simulink model "cable_driven_parallel_robot2022"  (R2022b)
settings: Solver=ode3  StartTime=0.0  StopTime=100  FixedStep=0.01  RelTol=1e-3
values from neighbouring files (symbols this model uses):
  cable_length = 1.2    [Model_Info.m]
  g = 9.81    [Model_Info.m]
  MP_H = 2    [Model_Info.m]
  MP_init_X = 0    [Model_Info.m]
  MP_init_Y = 0    [Model_Info.m]
  MP_init_Z = cable_length + (MP_H/2)    (= 2.2)    [Model_Info.m]
  MP_Ix = (MP_m/12)*(MP_W^2+MP_H^2)    (= 6.66666666667e-05)    [Model_Info.m]
  MP_Iy = (MP_m/12)*(MP_L^2+MP_H^2)    (= 6.66666666667e-05)    [Model_Info.m]
  MP_Iz = (MP_m/12)*(MP_L^2+MP_W^2)    (= 6.66666666667e-05)    [Model_Info.m]
  MP_L = 2    [Model_Info.m]
  MP_m = 0.0001    [Model_Info.m]
  MP_W = 2    [Model_Info.m]
  MR_init_X_L1 = -(MP_L/2)    (= -1)    [Model_Info.m]
  MR_init_X_L2 = (MP_L/2)    (= 1)    [Model_Info.m]
  MR_init_X_L3 = (MP_L/2)    (= 1)    [Model_Info.m]
  MR_init_X_L4 = -(MP_L/2)    (= -1)    [Model_Info.m]
  MR_init_Y_L1 = -(MP_W/2)    (= -1)    [Model_Info.m]
  MR_init_Y_L2 = -(MP_W/2)    (= -1)    [Model_Info.m]
  MR_init_Y_L3 = (MP_W/2)    (= 1)    [Model_Info.m]
  MR_init_Y_L4 = (MP_W/2)    (= 1)    [Model_Info.m]
  MR_init_Yaw_L1 = pi    (= 3.14159265359)    [Model_Info.m]
  MR_init_Yaw_L2 = 0    [Model_Info.m]
  MR_init_Yaw_L3 = 0    [Model_Info.m]
  MR_init_Yaw_L4 = pi    (= 3.14159265359)    [Model_Info.m]
  MR_Jr = (MR_m/12)*(MR_L^2+MR_W^2)    (= 0.333333333333)    [Model_Info.m]
  MR_m = 0.5    [Model_Info.m]
  MR_r = 2    [Model_Info.m]
  MR_WT = 2    [Model_Info.m]
  QR_Ax = 0.25*0    (= 0)    [Model_Info.m]
  QR_Ay = 0.25*0    (= 0)    [Model_Info.m]
  QR_Az = 0.25*0    (= 0)    [Model_Info.m]
  QR_b = 1.14*1e-7    (= 1.14e-07)    [Model_Info.m]
  QR_Ixx = 4.856*1e-3    (= 0.004856)    [Model_Info.m]
  QR_Iyy = 4.856*1e-3    (= 0.004856)    [Model_Info.m]
  QR_Izz = 8.801*1e-3    (= 0.008801)    [Model_Info.m]
  QR_K = 2.980*1e-6    (= 2.98e-06)    [Model_Info.m]
  QR_l = 0.225    [Model_Info.m]
  QR_m = 0.468    [Model_Info.m]
  QR_x0_U1 = -(MP_L/2)    (= -1)    [Model_Info.m]
  QR_x0_U2 = (MP_L/2)    (= 1)    [Model_Info.m]
  QR_x0_U3 = (MP_L/2)    (= 1)    [Model_Info.m]
  QR_x0_U4 = -(MP_L/2)    (= -1)    [Model_Info.m]
  QR_y0_U1 = -(MP_W/2)    (= -1)    [Model_Info.m]
  QR_y0_U2 = -(MP_W/2)    (= -1)    [Model_Info.m]
  QR_y0_U3 = (MP_W/2)    (= 1)    [Model_Info.m]
  QR_y0_U4 = (MP_W/2)    (= 1)    [Model_Info.m]
  QR_z0_U1 = 2*cable_length+(MP_H)    (= 4.4)    [Model_Info.m]
  QR_z0_U2 = 2*cable_length+(MP_H)    (= 4.4)    [Model_Info.m]
  QR_z0_U3 = 2*cable_length+(MP_H)    (= 4.4)    [Model_Info.m]
  QR_z0_U4 = 2*cable_length+(MP_H)    (= 4.4)    [Model_Info.m]
(part 12 of 12)

== matlab function cable_driven_parallel_robot2022/Target Wrench-Jacobian matrix/QuadRotor U4/Force Generator/QuadCopter Model ==
  data: vx input; x_ddot output size=1; vy input; vz input; phidot input; thetadot input; psidot input; y_ddot output size=1; z_ddot output size=1; phi input; theta input; psi input; constants input
function [x_ddot,y_ddot,z_ddot] = fcn(vx,vy,vz,phidot,thetadot,psidot, phi,theta,psi,constants)
m = constants(1);
g = constants(2);
Ixx = constants(3);
Iyy = constants(4);
Izz = constants(5);
l = constants(6);
K = constants(7);
b = constants(8);
Ax = constants(9);
Ay = constants(10);
Az = constants(11);
omega1 = constants(12);
omega2 = constants(13);
omega3 = constants(14);
omega4 = constants(15);
Tx = constants(16);
Ty = constants(17);
Tz = constants(18);
% x_ddot = (K*omega1^2*sin(phi)*sin(psi) - Ax*vx + K*omega2^2*sin(phi)*sin(psi) + K*omega3^2*sin(phi)*sin(psi) + K*omega4^2*sin(phi)*sin(psi) + K*omega1^2*cos(phi)*cos(psi)*sin(theta) + K*omega2^2*cos(phi)*cos(psi)*sin(theta) + K*omega3^2*cos(phi)*cos(psi)*sin(theta) + K*omega4^2*cos(phi)*cos(psi)*sin(theta))/m;
% y_ddot = -(Ay*vy + K*omega1^2*cos(psi)*sin(phi) + K*omega2^2*cos(psi)*sin(phi) + K*omega3^2*cos(psi)*sin(phi) + K*omega4^2*cos(psi)*sin(phi) - K*omega1^2*cos(phi)*sin(psi)*sin(theta) - K*omega2^2*cos(phi)*sin(psi)*sin(theta) - K*omega3^2*cos(phi)*sin(psi)*sin(theta) - K*omega4^2*cos(phi)*sin(psi)*sin(theta))/m;
% z_ddot = (K*cos(phi)*cos(theta)*omega1^2 + K*cos(phi)*cos(theta)*omega2^2 + K*cos(phi)*cos(theta)*omega3^2 + K*cos(phi)*cos(theta)*omega4^2 - Az*vz - g*m)/m;
% phi_ddot = (2*Ixx*Iyy*b*omega1^2*sin(theta) - 2*Ixx*Iyy*b*omega2^2*sin(theta) + 2*Ixx*Iyy*b*omega3^2*sin(theta) - 2*Ixx*Iyy*b*omega4^2*sin(theta) + 2*Iyy^3*psidot^2*cos(phi)*cos(theta)^4*sin(phi)^3 - 2*Iyy^3*psidot^2*cos(phi)*cos(theta)^4*sin(phi)^5 - 2*Iyy^3*psidot*thetadot*cos(theta)^3*sin(phi)^2 + 2*Iyy^3*psidot*thetadot*cos(theta)^3*sin(phi)^4 - 2*Iyy^3*psidot^2*cos(phi)^3*cos(theta)^4*sin(phi)^3 - Iyy^3*thetadot^2*sin(2*phi)*cos(theta)^2*sin(phi)^2 + Iyy^3*thetadot^2*sin(2*phi)*cos(theta)^2*sin(phi)^4 - Ixx*Iyy^2*thetadot^2*sin(2*phi)*sin(theta)^2 - 2*Iyy^2*K*l*omega2^2*cos(theta)^2*sin(phi)^2 + 2*Iyy^2*K*l*omega2^2*cos(theta)^2*sin(phi)^4 + 2*Iyy^2*K*l*omega4^2*cos(theta)^2*sin(phi)^2 - 2*Iyy^2*K*l*omega4^2*cos(theta)^2*sin(phi)^4 + 2*Ixx*Iyy^2*thetadot^2*cos(phi)*sin(phi)*sin(theta)^2 - 2*Ixx*Iyy*b*omega1^2*sin(phi)^2*sin(theta) + 2*Ixx*Iyy*b*omega2^2*sin(phi)^2*sin(theta) - 2*Ixx*Iyy*b*omega3^2*sin(phi)^2*sin(theta) + 2*Ixx*Iyy*b*omega4^2*sin(phi)^2*sin(theta) + 2*Ixx*Izz*b*omega1^2*sin(phi)^2*sin(theta) - 2*Ixx*Izz*b*omega2^2*sin(phi)^2*sin(theta) + 2*Ixx*Izz*b*omega3^2*sin(phi)^2*sin(theta) - 2*Ixx*Izz*b*omega4^2*sin(phi)^2*sin(theta) - 2*Ixx*Iyy^2*psidot*thetadot*cos(theta)*sin(theta)^2 + 2*Ixx^2*Iyy*psidot*thetadot*cos(theta)*sin(theta)^2 + 2*Ixx*Iyy^2*psidot*thetadot*sin(2*theta)*sin(theta) - 2*Ixx^2*Iyy*psidot*thetadot*sin(2*theta)*sin(theta) - 2*Iyy*Izz^2*psidot^2*cos(phi)^3*cos(theta)^4*sin(phi) - 2*Iyy^2*Izz*psidot^2*cos(phi)*cos(theta)^4*sin(phi)^3 + 2*Iyy^2*Izz*psidot^2*cos(phi)^3*cos(theta)^4*sin(phi) - 2*Iyy*Izz^2*psidot^2*cos(phi)*cos(theta)^4*sin(phi)^5 + 4*Iyy^2*Izz*psidot^2*cos(phi)*cos(theta)^4*sin(phi)^5 - 2*Ixx*Iyy^2*thetadot^2*cos(phi)*sin(phi)^3*sin(theta)^2 - 2*Ixx*Izz^2*thetadot^2*cos(phi)*sin(phi)^3*sin(theta)^2 + Ixx*Iyy*Izz*thetadot^2*sin(2*phi)*sin(theta)^2 + 6*Iyy^3*psidot*thetadot*cos(phi)^2*cos(theta)^3*sin(phi)^2 - 4*Iyy^3*psidot*thetadot*cos(phi)^2*cos(theta)^3*sin(phi)^4 - 4*Iyy^3*psidot*thetadot*cos(phi)^4*cos(theta)^3*sin(phi)^2 + 2*Iyy*Izz^2*psidot*thetadot*cos(phi)^2*cos(theta)^3 - 2*Iyy^2*Izz*psidot*thetadot*cos(phi)^2*cos(theta)^3 - 4*Iyy*Izz^2*psidot*thetadot*cos(phi)^4*cos(theta)^3 + 4*Iyy^2*Izz*psidot*thetadot*cos(phi)^4*cos(theta)^3 + 2*Ixx*Iyy^2*psidot*thetadot*cos(theta)^3*sin(phi)^2 - 2*Ixx*Iyy^2*psidot*thetadot*cos(theta)^3*sin(phi)^4 + 2*Iyy^2*Izz*psidot*thetadot*cos(theta)^3*sin(phi)^2 + 2*Iyy*Izz^2*psidot*thetadot*cos(theta)^3*sin(phi)^4 - 4*Iyy^2*Izz*psidot*thetadot*cos(theta)^3*sin(phi)^4 - 2*Ixx*Iyy*K*l*omega2^2*sin(theta)^2 + 2*Ixx*Iyy*K*l*omega4^2*sin(theta)^2 + Iyy^3*thetadot^2*sin(2*phi)*cos(phi)^2*cos(theta)^2*sin(phi)^2 - 2*Iyy*Izz^2*psidot^2*cos(phi)^3*cos(theta)^4*sin(phi)^3 + 4*Iyy^2*Izz*psidot^2*cos(phi)^3*cos(theta)^4*sin(phi)^3 + Iyy*Izz^2*thetadot^2*sin(2*phi)*cos(phi)^2*cos(theta)^2 - Iyy^2*Izz*thetadot^2*sin(2*phi)*cos(phi)^2*cos(theta)^2 + Iyy^2*Izz*thetadot^2*sin(2*phi)*cos(theta)^2*sin(phi)^2 + Iyy*Izz^2*thetadot^2*sin(2*phi)*cos(theta)^2*sin(phi)^4 - 2*Iyy^2*Izz*thetadot^2*sin(2*phi)*cos(theta)^2*sin(phi)^4 + Ixx*Iyy^2*thetadot^2*sin(2*phi)*sin(phi)^2*sin(theta)^2 + Ixx*Izz^2*thetadot^2*sin(2*phi)*sin(phi)^2*sin(theta)^2 + 2*Ixx*Iyy^2*phidot*thetadot*cos(theta)*sin(theta) + 2*Ixx^2*Iyy*phidot*thetadot*cos(theta)*sin(theta) + 2*Ixx*Iyy*K*l*omega2^2*sin(phi)^2*sin(theta)^2 - 2*Ixx*Iyy*K*l*omega4^2*sin(phi)^2*sin(theta)^2 - 2*Ixx*Izz*K*l*omega2^2*sin(phi)^2*sin(theta)^2 + 2*Ixx*Izz*K*l*omega4^2*sin(phi)^2*sin(theta)^2 - 2*Ixx*Iyy*Izz*thetadot^2*cos(phi)*sin(phi)*sin(theta)^2 + Iyy*Izz^2*thetadot^2*sin(2*phi)*cos(phi)^2*cos(theta)^2*sin(phi)^2 - 2*Iyy^2*Izz*thetadot^2*sin(2*phi)*cos(phi)^2*cos(theta)^2*sin(phi)^2 - 4*Ixx*Iyy^2*phidot*thetadot*cos(phi)^2*cos(theta)*sin(theta) - 2*Ixx*Iyy^2*phidot*thetadot*cos(theta)*sin(phi)^2*sin(theta) - 2*Ixx^2*Iyy*phidot*thetadot*cos(theta)*sin(phi)^2*sin(theta) - 2*Ixx*Izz^2*phidot*thetadot*cos(theta)*sin(phi)^2*sin(theta) + 2*Ixx^2*Izz*phidot*thetadot*cos(theta)*sin(phi)^2*sin(theta) + 2*Iyy^2*K*l*omega2^2*cos(phi)^2*cos(theta)^2*sin(phi)^2 - 2*Iyy^2*K*l*omega4^2*cos(phi)^2*cos(theta)^2*sin(phi)^2 + 2*Ixx*Iyy*Izz*psidot*thetadot*cos(theta)*sin(theta)^2 + 2*Ixx*Iyy^2*psidot^2*cos(phi)*cos(theta)^2*sin(phi)*sin(theta)^2 + 4*Ixx*Iyy*Izz*thetadot^2*cos(phi)*sin(phi)^3*sin(theta)^2 + 2*Ixx*Iyy*Izz*psidot*thetadot*cos(phi)^2*cos(theta)^3 + 2*Ixx*Iyy^2*psidot*thetadot*cos(theta)*sin(phi)^2*sin(theta)^2 - 2*Ixx^2*Iyy*psidot*thetadot*cos(theta)*sin(phi)^2*sin(theta)^2 + 2*Ixx*Izz^2*psidot*thetadot*cos(theta)*sin(phi)^2*sin(theta)^2 + 2*Ixx^2*Izz*psidot*thetadot*cos(theta)*sin(phi)^2*sin(theta)^2 + 2*Ixx*Iyy*Izz*psidot*thetadot*cos(theta)^3*sin(phi)^4 - 2*Ixx*Iyy^2*psidot*thetadot*sin(2*theta)*sin(phi)^2*sin(theta) + 2*Ixx^2*Iyy*psidot*thetadot*sin(2*theta)*sin(phi)^2*sin(theta) - 2*Ixx^2*Izz*psidot*thetadot*sin(2*theta)*sin(phi)^2*sin(theta) - 2*Ixx*Izz^2*psidot^2*cos(phi)*cos(theta)^2*sin(phi)^3*sin(theta)^2 - 2*Ixx*Izz^2*psidot^2*cos(phi)^3*cos(theta)^2*sin(phi)*sin(theta)^2 - 2*Ixx*Iyy*Izz*thetadot^2*sin(2*phi)*sin(phi)^2*sin(theta)^2 - 2*Ixx*Iyy*Izz*phidot*thetadot*cos(theta)*sin(theta) - 2*Iyy*Izz*K*l*omega2^2*cos(phi)^2*cos(theta)^2 + 2*Iyy*Izz*K*l*omega4^2*cos(phi)^2*cos(theta)^2 - 2*Ixx*Iyy^2*psidot*thetadot*cos(phi)^2*cos(theta)^3*sin(phi)^2 + 2*Iyy*Izz^2*psidot*thetadot*cos(phi)^2*cos(theta)^3*sin(phi)^2 - 8*Iyy^2*Izz*psidot*thetadot*cos(phi)^2*cos(theta)^3*sin(phi)^2 - 4*Iyy*Izz^2*psidot*thetadot*cos(phi)^2*cos(theta)^3*sin(phi)^4 - 4*Iyy*Izz^2*psidot*thetadot*cos(phi)^4*cos(theta)^3*sin(phi)^2 + 8*Iyy^2*Izz*psidot*thetadot*cos(phi)^2*cos(theta)^3*sin(phi)^4 + 8*Iyy^2*Izz*psidot*thetadot*cos(phi)^4*cos(theta)^3*sin(phi)^2 - 2*Iyy*Izz*K*l*omega2^2*cos(theta)^2*sin(phi)^4 + 2*Iyy*Izz*K*l*omega4^2*cos(theta)^2*sin(phi)^4 - 4*Ixx*Iyy^2*phidot*psidot*cos(phi)*cos(theta)^2*sin(phi)*sin(theta) + 2*Ixx^2*Iyy*phidot*psidot*cos(phi)*cos(theta)^2*sin(phi)*sin(theta) - 2*Ixx^2*Izz*phidot*psidot*cos(phi)*cos(theta)^2*sin(phi)*sin(theta) + 4*Ixx*Iyy*Izz*phidot*thetadot*cos(phi)^2*cos(theta)*sin(theta) + 4*Ixx*Iyy*Izz*phidot*thetadot*cos(theta)*sin(phi)^2*sin(theta) - 2*Iyy*Izz*K*l*omega2^2*cos(phi)^2*cos(theta)^2*sin(phi)^2 + 2*Iyy*Izz*K*l*omega4^2*cos(phi)^2*cos(theta)^2*sin(phi)^2 - 2*Ixx*Iyy*Izz*psidot^2*cos(phi)*cos(theta)^2*sin(phi)*sin(theta)^2 + 2*Ixx*Iyy^2*phidot*psidot*cos(phi)*cos(theta)^2*sin(phi)^3*sin(theta) + 2*Ixx*Iyy^2*phidot*psidot*cos(phi)^3*cos(theta)^2*sin(phi)*sin(theta) + 2*Ixx*Izz^2*phidot*psidot*cos(phi)*cos(theta)^2*sin(phi)^3*sin(theta) + 2*Ixx*Izz^2*phidot*psidot*cos(phi)^3*cos(theta)^2*sin(phi)*sin(theta) + 4*Ixx*Iyy^2*phidot*thetadot*cos(phi)^2*cos(theta)*sin(phi)^2*sin(theta) + 4*Ixx*Izz^2*phidot*thetadot*cos(phi)^2*cos(theta)*sin(phi)^2*sin(theta) - 4*Ixx*Iyy*Izz*psidot*thetadot*cos(theta)*sin(phi)^2*sin(theta)^2 + 2*Ixx*Iyy*Izz*psidot*thetadot*sin(2*theta)*sin(phi)^2*sin(theta) + 2*Ixx*Iyy*Izz*psidot^2*cos(phi)*cos(theta)^2*sin(phi)^3*sin(theta)^2 + 2*Ixx*Iyy*Izz*psidot^2*cos(phi)^3*cos(theta)^2*sin(phi)*sin(theta)^2 + 2*Ixx*Iyy*Izz*psidot*thetadot*cos(phi)^2*cos(theta)^3*sin(phi)^2 - Ixx^2*Iyy*psidot^2*sin(2*theta)*cos(phi)*cos(theta)*sin(phi)*sin(theta) + Ixx^2*Izz*psidot^2*sin(2*theta)*cos(phi)*cos(theta)*sin(phi)*sin(theta) - 4*Ixx*Iyy*Izz*phidot*psidot*cos(phi)*cos(theta)^2*sin(phi)^3*sin(theta) - 4*Ixx*Iyy*Izz*phidot*psidot*cos(phi)^3*cos(theta)^2*sin(phi)*sin(theta) - 8*Ixx*Iyy*Izz*phidot*thetadot*cos(phi)^2*cos(theta)*sin(phi)^2*sin(theta) + 2*Ixx*Iyy*K*l*omega1^2*cos(phi)*cos(theta)*sin(phi)*sin(theta) - 2*Ixx*Iyy*K*l*omega3^2*cos(phi)*cos(theta)*sin(phi)*sin(theta) - 2*Ixx*Izz*K*l*omega1^2*cos(phi)*cos(theta)*sin(phi)*sin(theta) + 2*Ixx*Izz*K*l*omega3^2*cos(phi)*cos(theta)*sin(phi)*sin(theta) - 2*Ixx*Iyy^2*phidot*thetadot*sin(2*phi)*cos(phi)*cos(theta)*sin(phi)*sin(theta) - 2*Ixx*Izz^2*phidot*thetadot*sin(2*phi)*cos(phi)*cos(theta)*sin(phi)*sin(theta) + 4*Ixx*Iyy*Izz*phidot*psidot*cos(phi)*cos(theta)^2*sin(phi)*sin(theta) + 4*Ixx*Iyy*Izz*phidot*thetadot*sin(2*phi)*cos(phi)*cos(theta)*sin(phi)*sin(theta))/(2*Ixx*cos(theta)^2*(- Iyy^2*cos(phi)^2*sin(phi)^2 - Iyy^2*sin(phi)^4 + Iyy^2*sin(phi)^2 + Izz*Iyy*cos(phi)^2*sin(phi)^2 + Izz*Iyy*cos(phi)^2 + Izz*Iyy*sin(phi)^4));
% theta_ddot = -(2*Izz^2*psidot^2*cos(phi)^4*cos(theta)^2*sin(theta) + 2*Iyy^2*thetadot^2*cos(phi)^2*sin(phi)^2*sin(theta) + 2*Izz^2*thetadot^2*cos(phi)^2*sin(phi)^2*sin(theta) + 2*Iyy^2*psidot^2*cos(theta)^2*sin(phi)^4*sin(theta) - 2*Izz^2*phidot*psidot*cos(phi)^4*cos(theta)^2 - 2*Iyy^2*phidot*psidot*cos(theta)^2*sin(phi)^4 + 2*Iyy*b*omega1^2*cos(phi)*sin(phi) - 2*Iyy*b*omega2^2*cos(phi)*sin(phi) + 2*Iyy*b*omega3^2*cos(phi)*sin(phi) - 2*Iyy*b*omega4^2*cos(phi)*sin(phi) - 2*Izz*b*omega1^2*cos(phi)*sin(phi) + 2*Izz*b*omega2^2*cos(phi)*sin(phi) - 2*Izz*b*omega3^2*cos(phi)*sin(phi) + 2*Izz*b*omega4^2*cos(phi)*sin(phi) - Ixx*Izz*psidot^2*sin(2*theta)*cos(phi)^2*cos(theta) - 4*Iyy*Izz*thetadot^2*cos(phi)^2*sin(phi)^2*sin(theta) - Ixx*Iyy*psidot^2*sin(2*theta)*cos(theta)*sin(phi)^2 + 2*Izz*K*l*omega1^2*cos(phi)^2*cos(theta) - 2*Izz*K*l*omega3^2*cos(phi)^2*cos(theta) + 2*Izz^2*phidot*thetadot*sin(2*phi)*cos(phi)^2*cos(theta) + 2*Ixx*Izz*phidot*psidot*cos(phi)^2*cos(theta)^2 + 2*Iyy*Izz*phidot*psidot*cos(phi)^4*cos(theta)^2 + 2*Iyy*K*l*omega1^2*cos(theta)*sin(phi)^2 - 2*Iyy*K*l*omega3^2*cos(theta)*sin(phi)^2 - 2*Iyy^2*phidot*thetadot*sin(2*phi)*cos(theta)*sin(phi)^2 + 2*Ixx*Iyy*phidot*psidot*cos(theta)^2*sin(phi)^2 + 2*Iyy*Izz*phidot*psidot*cos(theta)^2*sin(phi)^4 + 2*Iyy^2*psidot^2*cos(phi)^2*cos(theta)^2*sin(phi)^2*sin(theta) + 2*Izz^2*psidot^2*cos(phi)^2*cos(theta)^2*sin(phi)^2*sin(theta) + 2*Iyy^2*phidot*thetadot*cos(phi)*cos(theta)*sin(phi) + 2*Izz^2*phidot*thetadot*cos(phi)*cos(theta)*sin(phi) - 2*Iyy^2*phidot*psidot*cos(phi)^2*cos(theta)^2*sin(phi)^2 - 2*Izz^2*phidot*psidot*cos(phi)^2*cos(theta)^2*sin(phi)^2 - Iyy^2*thetadot^2*sin(2*phi)*cos(phi)*sin(phi)*sin(theta) - Izz^2*thetadot^2*sin(2*phi)*cos(phi)*sin(phi)*sin(theta) - 4*Iyy^2*phidot*thetadot*cos(phi)^3*cos(theta)*sin(phi) - 4*Izz^2*phidot*thetadot*cos(phi)^3*cos(theta)*sin(phi) + 2*Iyy^2*psidot*thetadot*sin(2*theta)*cos(phi)*sin(phi) - 2*Iyy*Izz*phidot*thetadot*sin(2*phi)*cos(phi)^2*cos(theta) + 2*Iyy*Izz*phidot*thetadot*sin(2*phi)*cos(theta)*sin(phi)^2 - 2*Iyy^2*psidot*thetadot*cos(phi)*cos(theta)*sin(phi)*sin(theta) - 2*Izz^2*psidot*thetadot*cos(phi)*cos(theta)*sin(phi)*sin(theta) + 2*Ixx*Iyy*phidot*thetadot*cos(phi)*cos(theta)*sin(phi) - 2*Ixx*Izz*phidot*thetadot*cos(phi)*cos(theta)*sin(phi) - 4*Iyy*Izz*phidot*thetadot*cos(phi)*cos(theta)*sin(phi) + 4*Iyy*Izz*phidot*psidot*cos(phi)^2*cos(theta)^2*sin(phi)^2 + 2*Iyy*Izz*thetadot^2*sin(2*phi)*cos(phi)*sin(phi)*sin(theta) + 8*Iyy*Izz*phidot*thetadot*cos(phi)^3*cos(theta)*sin(phi) - 2*Iyy*K*l*omega2^2*cos(phi)*sin(phi)*sin(theta) + 2*Iyy*K*l*omega4^2*cos(phi)*sin(phi)*sin(theta) + 2*Izz*K*l*omega2^2*cos(phi)*sin(phi)*sin(theta) - 2*Izz*K*l*omega4^2*cos(phi)*sin(phi)*sin(theta) - 2*Ixx*Iyy*psidot*thetadot*sin(2*theta)*cos(phi)*sin(phi) + 2*Ixx*Izz*psidot*thetadot*sin(2*theta)*cos(phi)*sin(phi) - 2*Iyy*Izz*psidot*thetadot*sin(2*theta)*cos(phi)*sin(phi) + 2*Ixx*Iyy*psidot*thetadot*cos(phi)*cos(theta)*sin(phi)*sin(theta) - 2*Ixx*Izz*psidot*thetadot*cos(phi)*cos(theta)*sin(phi)*sin(theta) + 4*Iyy*Izz*psidot*thetadot*cos(phi)*cos(theta)*sin(phi)*sin(theta))/(2*cos(theta)*(- Iyy^2*cos(phi)^2*sin(phi)^2 - Iyy^2*sin(phi)^4 + Iyy^2*sin(phi)^2 + Izz*Iyy*cos(phi)^2*sin(phi)^2 + Izz*Iyy*cos(phi)^2 + Izz*Iyy*sin(phi)^4));
% psi_ddot = (2*Iyy*b*omega1^2 - 2*Iyy*b*omega2^2 + 2*Iyy*b*omega3^2 - 2*Iyy*b*omega4^2 - Iyy^2*thetadot^2*sin(2*phi)*sin(theta) - 2*Iyy*b*omega1^2*sin(phi)^2 + 2*Iyy*b*omega2^2*sin(phi)^2 - 2*Iyy*b*omega3^2*sin(phi)^2 + 2*Iyy*b*omega4^2*sin(phi)^2 + 2*Izz*b*omega1^2*sin(phi)^2 - 2*Izz*b*omega2^2*sin(phi)^2 + 2*Izz*b*omega3^2*sin(phi)^2 - 2*Izz*b*omega4^2*sin(phi)^2 + 2*Iyy^2*psidot*thetadot*sin(2*theta) + 2*Iyy^2*phidot*thetadot*cos(theta) - 2*Iyy^2*phidot*thetadot*cos(theta)*sin(phi)^2 - 2*Izz^2*phidot*thetadot*cos(theta)*sin(phi)^2 - 2*Iyy*K*l*omega2^2*sin(theta) + 2*Iyy*K*l*omega4^2*sin(theta) - 2*Ixx*Iyy*psidot*thetadot*sin(2*theta) + Iyy^2*thetadot^2*sin(2*phi)*sin(phi)^2*sin(theta) + Izz^2*thetadot^2*sin(2*phi)*sin(phi)^2*sin(theta) - 2*Iyy^2*psidot*thetadot*sin(2*theta)*sin(phi)^2 + 2*Iyy^2*thetadot^2*cos(phi)*sin(phi)*sin(theta) - 2*Iyy^2*psidot*thetadot*cos(theta)*sin(theta) + 2*Ixx*Iyy*phidot*thetadot*cos(theta) - 2*Iyy*Izz*phidot*thetadot*cos(theta) - 2*Iyy^2*thetadot^2*cos(phi)*sin(phi)^3*sin(theta) - 2*Izz^2*thetadot^2*cos(phi)*sin(phi)^3*sin(theta) + Iyy*Izz*thetadot^2*sin(2*phi)*sin(theta) - 4*Iyy^2*phidot*thetadot*cos(phi)^2*cos(theta) - 2*Izz^2*psidot^2*cos(phi)*cos(theta)^2*sin(phi)^3*sin(theta) - 2*Izz^2*psidot^2*cos(phi)^3*cos(theta)^2*sin(phi)*sin(theta) - 2*Iyy*Izz*thetadot^2*sin(2*phi)*sin(phi)^2*sin(theta) + 2*Iyy^2*phidot*psidot*cos(phi)*cos(theta)^2*sin(phi)^3 + 2*Iyy^2*phidot*psidot*cos(phi)^3*cos(theta)^2*sin(phi) + 2*Izz^2*phidot*psidot*cos(phi)*cos(theta)^2*sin(phi)^3 + 2*Izz^2*phidot*psidot*cos(phi)^3*cos(theta)^2*sin(phi) + 4*Iyy^2*phidot*thetadot*cos(phi)^2*cos(theta)*sin(phi)^2 + 4*Izz^2*phidot*thetadot*cos(phi)^2*cos(theta)*sin(phi)^2 + 2*Iyy*K*l*omega2^2*sin(phi)^2*sin(theta) - 2*Iyy*K*l*omega4^2*sin(phi)^2*sin(theta) - 2*Izz*K*l*omega2^2*sin(phi)^2*sin(theta) + 2*Izz*K*l*omega4^2*sin(phi)^2*sin(theta) + 2*Ixx*Iyy*psidot*thetadot*sin(2*theta)*sin(phi)^2 - 2*Ixx*Izz*psidot*thetadot*sin(2*theta)*sin(phi)^2 + 2*Iyy*Izz*psidot*thetadot*sin(2*theta)*sin(phi)^2 - 2*Iyy*Izz*thetadot^2*cos(phi)*sin(phi)*sin(theta) + 2*Ixx*Iyy*psidot*thetadot*cos(theta)*sin(theta) + 2*Iyy*Izz*psidot*thetadot*cos(theta)*sin(theta) + 2*Iyy^2*psidot^2*cos(phi)*cos(theta)^2*sin(phi)*sin(theta) + 4*Iyy*Izz*thetadot^2*cos(phi)*sin(phi)^3*sin(theta) - 4*Iyy^2*phidot*psidot*cos(phi)*cos(theta)^2*sin(phi) + 4*Iyy*Izz*phidot*thetadot*cos(phi)^2*cos(theta) + 2*Iyy^2*psidot*thetadot*cos(theta)*sin(phi)^2*sin(theta) + 2*Izz^2*psidot*thetadot*cos(theta)*sin(phi)^2*sin(theta) - 2*Ixx*Iyy*phidot*thetadot*cos(theta)*sin(phi)^2 + 2*Ixx*Izz*phidot*thetadot*cos(theta)*sin(phi)^2 + 4*Iyy*Izz*phidot*thetadot*cos(theta)*sin(phi)^2 - 4*Iyy*Izz*phidot*psidot*cos(phi)*cos(theta)^2*sin(phi)^3 - 4*Iyy*Izz*phidot*psidot*cos(phi)^3*cos(theta)^2*sin(phi) - 8*Iyy*Izz*phidot*thetadot*cos(phi)^2*cos(theta)*sin(phi)^2 - Ixx*Iyy*psidot^2*sin(2*theta)*cos(phi)*cos(theta)*sin(phi) + Ixx*Izz*psidot^2*sin(2*theta)*cos(phi)*cos(theta)*sin(phi) - 2*Iyy*Izz*psidot^2*cos(phi)*cos(theta)^2*sin(phi)*sin(theta) + 2*Iyy*K*l*omega1^2*cos(phi)*cos(theta)*sin(phi) - 2*Iyy*K*l*omega3^2*cos(phi)*cos(theta)*sin(phi) - 2*Izz*K*l*omega1^2*cos(phi)*cos(theta)*sin(phi) + 2*Izz*K*l*omega3^2*cos(phi)*cos(theta)*sin(phi) - 2*Iyy^2*phidot*thetadot*sin(2*phi)*cos(phi)*cos(theta)*sin(phi) - 2*Izz^2*phidot*thetadot*sin(2*phi)*cos(phi)*cos(theta)*sin(phi) + 2*Ixx*Iyy*phidot*psidot*cos(phi)*cos(theta)^2*sin(phi) - 2*Ixx*Izz*phidot*psidot*cos(phi)*cos(theta)^2*sin(phi) + 4*Iyy*Izz*phidot*psidot*cos(phi)*cos(theta)^2*sin(phi) - 2*Ixx*Iyy*psidot*thetadot*cos(theta)*sin(phi)^2*sin(theta) + 2*Ixx*Izz*psidot*thetadot*cos(theta)*sin(phi)^2*sin(theta) - 4*Iyy*Izz*psidot*thetadot*cos(theta)*sin(phi)^2*sin(theta) + 2*Iyy*Izz*psidot^2*cos(phi)*cos(theta)^2*sin(phi)^3*sin(theta) + 2*Iyy*Izz*psidot^2*cos(phi)^3*cos(theta)^2*sin(phi)*sin(theta) + 4*Iyy*Izz*phidot*thetadot*sin(2*phi)*cos(phi)*cos(theta)*sin(phi))/(2*cos(theta)^2*(- Iyy^2*cos(phi)^2*sin(phi)^2 - Iyy^2*sin(phi)^4 + Iyy^2*sin(phi)^2 + Izz*Iyy*cos(phi)^2*sin(phi)^2 + Izz*Iyy*cos(phi)^2 + Izz*Iyy*sin(phi)^4));
x_ddot =  (K*omega1^2*sin(phi)*sin(psi) - Ax*vx - Tx + K*omega2^2*sin(phi)*sin(psi) + K*omega3^2*sin(phi)*sin(psi) + K*omega4^2*sin(phi)*sin(psi) + K*omega1^2*cos(phi)*cos(psi)*sin(theta) + K*omega2^2*cos(phi)*cos(psi)*sin(theta) + K*omega3^2*cos(phi)*cos(psi)*sin(theta) + K*omega4^2*cos(phi)*cos(psi)*sin(theta))/m;
y_ddot = -(Ty + Ay*vy + K*omega1^2*cos(psi)*sin(phi) + K*omega2^2*cos(psi)*sin(phi) + K*omega3^2*cos(psi)*sin(phi) + K*omega4^2*cos(psi)*sin(phi) - K*omega1^2*cos(phi)*sin(psi)*sin(theta) - K*omega2^2*cos(phi)*sin(psi)*sin(theta) - K*omega3^2*cos(phi)*sin(psi)*sin(theta) - K*omega4^2*cos(phi)*sin(psi)*sin(theta))/m;
z_ddot = (K*cos(phi)*cos(theta)*omega1^2 + K*cos(phi)*cos(theta)*omega2^2 + K*cos(phi)*cos(theta)*omega3^2 + K*cos(phi)*cos(theta)*omega4^2 - Tz - Az*vz - g*m)/m;

end

== matlab function cable_driven_parallel_robot2022/Target Wrench-Jacobian matrix/Moving Platform/Moving Platform/QR Force Generator ==
  data: mass input; Fx output; Fy output; Fz output
function [Fx,Fy,Fz] = fcn(mass)
g = 9.81;

Fx = 0;
Fy = 0;
Fz = -mass*g; 
    
end

== matlab function cable_driven_parallel_robot2022/Target Wrench-Jacobian matrix/2 Wheels Diffrential Mobile Robot L1/Transform ==
  data: roll input; pitch input; yaw input; MP_X input; MP_Y input; MP_Z input; MP_L1_X output; MP_L1_Y output; MP_L1_Z output; L input; W input; H input
function [MP_L1_X,MP_L1_Y,MP_L1_Z] = fcn(roll,pitch,yaw,MP_X,MP_Y,MP_Z,L,W,H)

MP_C = [1  0  0  MP_X; ... 
        0  1  0  MP_Y; ...
        0  0  1  MP_Z; ...
        0  0  0   1];

R_x = [1      0          0          0; ...
       0  cos(roll) -sin(roll)      0; ...
       0  sin(roll)  cos(roll)      0; ...
       0      0          0          1];
   
R_y = [cos(pitch)  0   sin(pitch)   0; ...
          0        1       0        0; ...
      -sin(pitch)  0   cos(pitch)   0; ...
          0        0       0        1];
   
R_z = [cos(yaw) -sin(yaw)  0        0; ...
       sin(yaw)  cos(yaw)  0        0; ...
         0           0     1        0; ...
         0           0     0        1];

R = MP_C*R_z*R_y*R_x;

Out = R* ([-(L/2);-(W/2) ;-(H/2);1]);
MP_L1_X = Out(1);
MP_L1_Y = Out(2);
MP_L1_Z = Out(3);

== matlab function cable_driven_parallel_robot2022/Target Wrench-Jacobian matrix/2 Wheels Diffrential Mobile Robot L2/Transform ==
  data: roll input; pitch input; yaw input; MP_X input; MP_Y input; MP_Z input; MP_L2_X output; MP_L2_Y output; MP_L2_Z output; L input; W input; H input
function [MP_L2_X,MP_L2_Y,MP_L2_Z] = fcn(roll,pitch,yaw,MP_X,MP_Y,MP_Z,L,W,H)

MP_C = [1  0  0  MP_X; ... 
        0  1  0  MP_Y; ...
        0  0  1  MP_Z; ...
        0  0  0   1];

R_x = [1      0          0          0; ...
       0  cos(roll) -sin(roll)      0; ...
       0  sin(roll)  cos(roll)      0; ...
       0      0          0          1];
   
R_y = [cos(pitch)  0   sin(pitch)   0; ...
          0        1       0        0; ...
      -sin(pitch)  0   cos(pitch)   0; ...
          0        0       0        1];
   
R_z = [cos(yaw) -sin(yaw)  0        0; ...
       sin(yaw)  cos(yaw)  0        0; ...
         0           0     1        0; ...
         0           0     0        1];

R = MP_C*R_z*R_y*R_x;

Out = R* ([(L/2);-(W/2);-(H/2);1]);
MP_L2_X = Out(1);
MP_L2_Y = Out(2);
MP_L2_Z = Out(3);

== matlab function cable_driven_parallel_robot2022/Target Wrench-Jacobian matrix/2 Wheels Diffrential Mobile Robot L3/Transform ==
  data: roll input; pitch input; yaw input; MP_X input; MP_Y input; MP_Z input; MP_L3_X output; MP_L3_Y output; MP_L3_Z output; L input; W input; H input
function [MP_L3_X,MP_L3_Y,MP_L3_Z] = fcn(roll,pitch,yaw,MP_X,MP_Y,MP_Z,L,W,H)

MP_C = [1  0  0  MP_X; ... 
        0  1  0  MP_Y; ...
        0  0  1  MP_Z; ...
        0  0  0   1];

R_x = [1      0          0          0; ...
       0  cos(roll) -sin(roll)      0; ...
       0  sin(roll)  cos(roll)      0; ...
       0      0          0          1];
   
R_y = [cos(pitch)  0   sin(pitch)   0; ...
          0        1       0        0; ...
      -sin(pitch)  0   cos(pitch)   0; ...
          0        0       0        1];
   
R_z = [cos(yaw) -sin(yaw)  0        0; ...
       sin(yaw)  cos(yaw)  0        0; ...
         0           0     1        0; ...
         0           0     0        1];

R = MP_C*R_z*R_y*R_x;

Out = R* ([(L/2);+(W/2);-(H/2);1]);
MP_L3_X = Out(1);
MP_L3_Y = Out(2);
MP_L3_Z = Out(3);

== matlab function cable_driven_parallel_robot2022/Target Wrench-Jacobian matrix/2 Wheels Diffrential Mobile Robot L4/Transform ==
  data: roll input; pitch input; yaw input; MP_X input; MP_Y input; MP_Z input; MP_L4_X output; MP_L4_Y output; MP_L4_Z output; L input; W input; H input
function [MP_L4_X,MP_L4_Y,MP_L4_Z] = fcn(roll,pitch,yaw,MP_X,MP_Y,MP_Z,L,W,H)

MP_C = [1  0  0  MP_X; ... 
        0  1  0  MP_Y; ...
        0  0  1  MP_Z; ...
        0  0  0   1];

R_x = [1      0          0          0; ...
       0  cos(roll) -sin(roll)      0; ...
       0  sin(roll)  cos(roll)      0; ...
       0      0          0          1];
   
R_y = [cos(pitch)  0   sin(pitch)   0; ...
          0        1       0        0; ...
      -sin(pitch)  0   cos(pitch)   0; ...
          0        0       0        1];
   
R_z = [cos(yaw) -sin(yaw)  0        0; ...
       sin(yaw)  cos(yaw)  0        0; ...
         0           0     1        0; ...
         0           0     0        1];

R = MP_C*R_z*R_y*R_x;

Out = R* ([-(L/2);+(W/2);-(H/2);1]);
MP_L4_X = Out(1);
MP_L4_Y = Out(2);
MP_L4_Z = Out(3);

== matlab function cable_driven_parallel_robot2022/Actuators-CableTension-MovingPlatform/Moving Platform/Moving Platform/Moving Platform ==
  settings: updateMethod=DISCRETE
  data: Tx_U1 input; Ty_U1 input; Tz_U1 input; Tx_U2 input; Ty_U2 input; Tz_U2 input; Tx_U3 input; Ty_U3 input; Tz_U3 input; Tx_U4 input; Ty_U4 input; Tz_U4 input; Tx_L1 input; Ty_L1 input; Tz_L1 input; ax output; Tx_L2 input; Ty_L2 input; Tz_L2 input; ay output; Tx_L3 input; Ty_L3 input; Tz_L3 input; Tx_L4 input; Ty_L4 input; Tz_L4 input; m input; Ix input; Iy input; Iz input; gx input; gy input; gz input; L input; W input; H input; az output; alpha_x output; alpha_y output; alpha_z output
function [ax,ay,az,alpha_x,alpha_y,alpha_z] = fcn(Tx_U1,Ty_U1,Tz_U1,Tx_U2,Ty_U2,Tz_U2,Tx_U3,Ty_U3,Tz_U3,Tx_U4,Ty_U4,Tz_U4,Tx_L1,Ty_L1,Tz_L1,Tx_L2,Ty_L2,Tz_L2,Tx_L3,Ty_L3,Tz_L3,Tx_L4,Ty_L4,Tz_L4,m,Ix,Iy,Iz,gx,gy,gz,L,W,H)



ax=(Tx_U1+Tx_U2+Tx_U3+Tx_U4+Tx_L1+Tx_L2+Tx_L3+Tx_L4-m*gx)/m;

ay=(Ty_U1+Ty_U2+Ty_U3+Ty_U4+Ty_L1+Ty_L2+Ty_L3+Ty_L4-m*gy)/m;

az=(Tz_U1+Tz_U2+Tz_U3+Tz_U4+Tz_L1+Tz_L2+Tz_L3+Tz_L4-m*gz)/m;

 alpha_x =((Ty_L1+Ty_L2+Ty_L3+Ty_L4)* (H/2)...
          -(Ty_U1+Ty_U2+Ty_U3+Ty_U4)* (H/2)...
          +(Tz_U3+Tz_U4+Tz_L3+Tz_L4)* (W/2)...
          -(Tz_U1+Tz_U2+Tz_L1+Tz_L2)* (W/2))/Ix;
      
 alpha_y =((Tx_U1+Tx_U2+Tx_U3+Tx_U4)* (H/2)...
          -(Tx_L1+Tx_L2+Tx_L3+Tx_L4)* (H/2)...
          +(Tz_U1+Tz_U4+Tz_L1+Tz_L4)* (L/2)...
          -(Tz_U2+Tz_U3+Tz_L2+Tz_L3)* (L/2))/Iy;
      
 alpha_z =((Tx_U1+Tx_U2+Tx_L1+Tx_L2)* (W/2)...
          -(Tx_U3+Tx_U4+Tx_L3+Tx_L4)* (W/2)...
          +(Ty_U2+Ty_U3+Ty_L2+Ty_L3)* (L/2)...
          -(Ty_U1+Ty_U4+Ty_L1+Ty_L4)* (L/2))/Iz;

== matlab function cable_driven_parallel_robot2022/Target Wrench-Jacobian matrix/QuadRotor U1/Transform ==
  data: roll input; pitch input; yaw input; MP_X input; MP_Y input; MP_Z input; MP_U1_X output; MP_U1_Y output; MP_U1_Z output; L input; W input; H input
function [MP_U1_X,MP_U1_Y,MP_U1_Z] = fcn(roll,pitch,yaw,MP_X,MP_Y,MP_Z,L,W,H)

MP_C = [1  0  0  MP_X; ... 
        0  1  0  MP_Y; ...
        0  0  1  MP_Z; ...
        0  0  0   1];

R_x = [1      0          0          0; ...
       0  cos(roll) -sin(roll)      0; ...
       0  sin(roll)  cos(roll)      0; ...
       0      0          0          1];
   
R_y = [cos(pitch)  0   sin(pitch)   0; ...
          0        1       0        0; ...
      -sin(pitch)  0   cos(pitch)   0; ...
          0        0       0        1];
   
R_z = [cos(yaw) -sin(yaw)  0        0; ...
       sin(yaw)  cos(yaw)  0        0; ...
         0           0     1        0; ...
         0           0     0        1];

R = MP_C*R_z*R_y*R_x;

Out = R* ([-(L/2);-(W/2) ;(H/2);1]);
MP_U1_X = Out(1);
MP_U1_Y = Out(2);
MP_U1_Z = Out(3);

== matlab function cable_driven_parallel_robot2022/Target Wrench-Jacobian matrix/QuadRotor U2/Transform ==
  data: roll input; pitch input; yaw input; MP_X input; MP_Y input; MP_Z input; MP_U2_X output; MP_U2_Y output; MP_U2_Z output; L input; W input; H input
function [MP_U2_X,MP_U2_Y,MP_U2_Z] = fcn(roll,pitch,yaw,MP_X,MP_Y,MP_Z,L,W,H)

MP_C = [1  0  0  MP_X; ... 
        0  1  0  MP_Y; ...
        0  0  1  MP_Z; ...
        0  0  0   1];

R_x = [1      0          0          0; ...
       0  cos(roll) -sin(roll)      0; ...
       0  sin(roll)  cos(roll)      0; ...
       0      0          0          1];
   
R_y = [cos(pitch)  0   sin(pitch)   0; ...
          0        1       0        0; ...
      -sin(pitch)  0   cos(pitch)   0; ...
          0        0       0        1];
   
R_z = [cos(yaw) -sin(yaw)  0        0; ...
       sin(yaw)  cos(yaw)  0        0; ...
         0           0     1        0; ...
         0           0     0        1];

R = MP_C*R_z*R_y*R_x;

Out = R* ([(L/2);-(W/2);(H/2);1]);
MP_U2_X = Out(1);
MP_U2_Y = Out(2);
MP_U2_Z = Out(3);

== matlab function cable_driven_parallel_robot2022/Target Wrench-Jacobian matrix/QuadRotor U3/Transform ==
  data: roll input; pitch input; yaw input; MP_X input; MP_Y input; MP_Z input; MP_U3_X output; MP_U3_Y output; MP_U3_Z output; L input; W input; H input
function [MP_U3_X,MP_U3_Y,MP_U3_Z] = fcn(roll,pitch,yaw,MP_X,MP_Y,MP_Z,L,W,H)
MP_C = [1  0  0  MP_X; ... 
        0  1  0  MP_Y; ...
        0  0  1  MP_Z; ...
        0  0  0   1];

R_x = [1      0          0          0; ...
       0  cos(roll) -sin(roll)      0; ...
       0  sin(roll)  cos(roll)      0; ...
       0      0          0          1];
   
R_y = [cos(pitch)  0   sin(pitch)   0; ...
          0        1       0        0; ...
      -sin(pitch)  0   cos(pitch)   0; ...
          0        0       0        1];
   
R_z = [cos(yaw) -sin(yaw)  0        0; ...
       sin(yaw)  cos(yaw)  0        0; ...
         0           0     1        0; ...
         0           0     0        1];

R = MP_C*R_z*R_y*R_x;

Out = R* ([(L/2);+(W/2);(H/2);1]);
MP_U3_X = Out(1);
MP_U3_Y = Out(2);
MP_U3_Z = Out(3);

== matlab function cable_driven_parallel_robot2022/Target Wrench-Jacobian matrix/QuadRotor U4/Transform ==
  data: roll input; pitch input; yaw input; MP_X input; MP_Y input; MP_Z input; MP_U4_X output; MP_U4_Y output; MP_U4_Z output; L input; W input; H input
function [MP_U4_X,MP_U4_Y,MP_U4_Z] = fcn(roll,pitch,yaw,MP_X,MP_Y,MP_Z,L,W,H)

MP_C = [1  0  0  MP_X; ... 
        0  1  0  MP_Y; ...
        0  0  1  MP_Z; ...
        0  0  0   1];

R_x = [1      0          0          0; ...
       0  cos(roll) -sin(roll)      0; ...
       0  sin(roll)  cos(roll)      0; ...
       0      0          0          1];
   
R_y = [cos(pitch)  0   sin(pitch)   0; ...
          0        1       0        0; ...
      -sin(pitch)  0   cos(pitch)   0; ...
          0        0       0        1];
   
R_z = [cos(yaw) -sin(yaw)  0        0; ...
       sin(yaw)  cos(yaw)  0        0; ...
         0           0     1        0; ...
         0           0     0        1];

R = MP_C*R_z*R_y*R_x;

Out = R* ([-(L/2);+(W/2);(H/2);1]);
MP_U4_X = Out(1);
MP_U4_Y = Out(2);
MP_U4_Z = Out(3);

== matlab function cable_driven_parallel_robot2022/Target Wrench-Jacobian matrix/Subsystem/MATLAB Function2 ==
  data: QR_Fz_U1 input; QR_Tz_U1 output; QR_Fz_U2 input; QR_Fz_U3 input; QR_Fz_U4 input; MP_Fz input; MR_Fz_L1 input; MR_Fz_L2 input; MR_Fz_L3 input; MR_Fz_L4 input; isTension input; QR_z_U1 input; QR_z_U2 input; QR_z_U3 input; QR_z_U4 input; MP_U1 input; MP_U2 input; MP_U3 input; MP_U4 input; MP_L1 input; MP_L2 input; MP_L3 input; MP_L4 input; MR_z_L1 input; MR_z_L2 input; MR_z_L3 input; MR_z_L4 input; QR_m input; MP_m input; MR_m input; QR_Tz_U2 output; QR_Tz_U3 output; QR_Tz_U4 output; MR_Tz_L1 output; MR_Tz_L2 output; MR_Tz_L3 output; MR_Tz_L4 output
function [QR_Tz_U1,QR_Tz_U2,QR_Tz_U3,QR_Tz_U4,MR_Tz_L1,MR_Tz_L2,MR_Tz_L3,MR_Tz_L4] = fcn(QR_Fz_U1,QR_Fz_U2,QR_Fz_U3,QR_Fz_U4,MP_Fz,MR_Fz_L1,MR_Fz_L2,MR_Fz_L3,MR_Fz_L4,isTension,QR_z_U1,QR_z_U2,QR_z_U3,QR_z_U4,MP_U1,MP_U2,MP_U3,MP_U4,MP_L1,MP_L2,MP_L3,MP_L4,MR_z_L1,MR_z_L2,MR_z_L3,MR_z_L4,QR_m,MP_m,MR_m)

MP_Fz = MP_Fz*or(sum(isTension),0);
gnd=[MR_z_L1<=0, MR_z_L2<=0, MR_z_L3<=0,MR_z_L4<=0];
Ngnd=[MR_z_L1>0, MR_z_L2>0, MR_z_L3>0,MR_z_L4>0];

up_F=QR_Fz_U1+QR_Fz_U2+QR_Fz_U3+QR_Fz_U4+MP_Fz+Ngnd(1)*MR_Fz_L1+Ngnd(2)*MR_Fz_L2+Ngnd(3)*MR_Fz_L3+Ngnd(4)*MR_Fz_L4;
down_F= -(gnd(1)*MR_Fz_L1+gnd(2)*MR_Fz_L2+gnd(3)*MR_Fz_L3+gnd(4)*MR_Fz_L4);

GNDcheck = up_F-down_F;

if  GNDcheck>=0     
    Fz_Total = QR_Fz_U1+QR_Fz_U2+QR_Fz_U3+QR_Fz_U4+MP_Fz+MR_Fz_L1+MR_Fz_L2+MR_Fz_L3+MR_Fz_L4;
    if Fz_Total==0
        az = 0;
    else

      m_Total = (isTension(1)+isTension(2)+isTension(3)+isTension(4))*QR_m +...
                                               (or(sum(isTension),0))*MP_m +...
                (isTension(5)+isTension(6)+isTension(7)+isTension(8))*MR_m;
      
      az = Fz_Total/m_Total;
    end
elseif ((QR_Fz_U1+QR_Fz_U2+QR_Fz_U3+QR_Fz_U4+MP_Fz)>=0)

    az = 0;
    MR_Fz_L1 = -(up_F)/(sum(gnd));
    MR_Fz_L2 = -(up_F)/(sum(gnd));
    MR_Fz_L3 = -(up_F)/(sum(gnd));
    MR_Fz_L4 = -(up_F)/(sum(gnd));

else
    Fz_Total = QR_Fz_U1+QR_Fz_U2+QR_Fz_U3+QR_Fz_U4+MP_Fz;
    if Fz_Total==0
        az = 0;
    else

      m_Total = (isTension(1)+isTension(2)+isTension(3)+isTension(4))*QR_m +...
                                               (or(sum(isTension),0))*MP_m +...
                (isTension(5)+isTension(6)+isTension(7)+isTension(8))*MR_m;
      
      az = Fz_Total/m_Total;
    end
    MR_Fz_L1 = 0;
    MR_Fz_L2 = 0;
    MR_Fz_L3 = 0;
    MR_Fz_L4 = 0;
end
     
QR_Tz_U1 = max(((MP_U1(3)-QR_z_U1)/(abs(MP_U1(3)-QR_z_U1)))*(QR_m*az - QR_Fz_U1),0)*isTension(1);
QR_Tz_U2 = max(((MP_U2(3)-QR_z_U2)/(abs(MP_U2(3)-QR_z_U2)))*(QR_m*az - QR_Fz_U2),0)*isTension(2);
QR_Tz_U3 = max(((MP_U3(3)-QR_z_U3)/(abs(MP_U3(3)-QR_z_U3)))*(QR_m*az - QR_Fz_U3),0)*isTension(3);
QR_Tz_U4 = max(((MP_U4(3)-QR_z_U4)/(abs(MP_U4(3)-QR_z_U4)))*(QR_m*az - QR_Fz_U4),0)*isTension(4);
MR_Tz_L1 = max(((MP_L1(3)-MR_z_L1)/(abs(MP_L1(3)-MR_z_L1)))*(MR_m*az - MR_Fz_L1),0)*isTension(5);
MR_Tz_L2 = max(((MP_L2(3)-MR_z_L2)/(abs(MP_L2(3)-MR_z_L2)))*(MR_m*az - MR_Fz_L2),0)*isTension(6);
MR_Tz_L3 = max(((MP_L3(3)-MR_z_L3)/(abs(MP_L3(3)-MR_z_L3)))*(MR_m*az - MR_Fz_L3),0)*isTension(7);
MR_Tz_L4 = max(((MP_L4(3)-MR_z_L4)/(abs(MP_L4(3)-MR_z_L4)))*(MR_m*az - MR_Fz_L4),0)*isTension(8);
end

== matlab function cable_driven_parallel_robot2022/Target Wrench-Jacobian matrix/Subsystem/Transformer/Transform ==
  data: roll input; pitch input; yaw input; MP_X input; MP_Y input; MP_Z input; MP_U1_X output; MP_U1_Y output; MP_U1_Z output; L input; W input; H input
function [MP_U1_X,MP_U1_Y,MP_U1_Z] = fcn(roll,pitch,yaw,MP_X,MP_Y,MP_Z,L,W,H)

MP_C = [1  0  0  MP_X; ... 
        0  1  0  MP_Y; ...
        0  0  1  MP_Z; ...
        0  0  0   1];

R_x = [1      0          0          0; ...
       0  cos(roll) -sin(roll)      0; ...
       0  sin(roll)  cos(roll)      0; ...
       0      0          0          1];
   
R_y = [cos(pitch)  0   sin(pitch)   0; ...
          0        1       0        0; ...
      -sin(pitch)  0   cos(pitch)   0; ...
          0        0       0        1];
   
R_z = [cos(yaw) -sin(yaw)  0        0; ...
       sin(yaw)  cos(yaw)  0        0; ...
         0           0     1        0; ...
         0           0     0        1];

R = MP_C*R_z*R_y*R_x;

Out = R* ([-(L/2);-(W/2) ;(H/2);1]);
MP_U1_X = Out(1);
MP_U1_Y = Out(2);
MP_U1_Z = Out(3);

== matlab function cable_driven_parallel_robot2022/Target Wrench-Jacobian matrix/Subsystem/Transformer/Transform1 ==
  data: roll input; pitch input; yaw input; MP_X input; MP_Y input; MP_Z input; MP_U2_X output; MP_U2_Y output; MP_U2_Z output; L input; W input; H input
function [MP_U2_X,MP_U2_Y,MP_U2_Z] = fcn(roll,pitch,yaw,MP_X,MP_Y,MP_Z,L,W,H)

MP_C = [1  0  0  MP_X; ... 
        0  1  0  MP_Y; ...
        0  0  1  MP_Z; ...
        0  0  0   1];

R_x = [1      0          0          0; ...
       0  cos(roll) -sin(roll)      0; ...
       0  sin(roll)  cos(roll)      0; ...
       0      0          0          1];
   
R_y = [cos(pitch)  0   sin(pitch)   0; ...
          0        1       0        0; ...
      -sin(pitch)  0   cos(pitch)   0; ...
          0        0       0        1];
   
R_z = [cos(yaw) -sin(yaw)  0        0; ...
       sin(yaw)  cos(yaw)  0        0; ...
         0           0     1        0; ...
         0           0     0        1];

R = MP_C*R_z*R_y*R_x;

Out = R* ([(L/2);-(W/2);(H/2);1]);
MP_U2_X = Out(1);
MP_U2_Y = Out(2);
MP_U2_Z = Out(3);

== matlab function cable_driven_parallel_robot2022/Target Wrench-Jacobian matrix/Subsystem/Transformer/Transform2 ==
  data: roll input; pitch input; yaw input; MP_X input; MP_Y input; MP_Z input; MP_U3_X output; MP_U3_Y output; MP_U3_Z output; L input; W input; H input
function [MP_U3_X,MP_U3_Y,MP_U3_Z] = fcn(roll,pitch,yaw,MP_X,MP_Y,MP_Z,L,W,H)
MP_C = [1  0  0  MP_X; ... 
        0  1  0  MP_Y; ...
        0  0  1  MP_Z; ...
        0  0  0   1];

R_x = [1      0          0          0; ...
       0  cos(roll) -sin(roll)      0; ...
       0  sin(roll)  cos(roll)      0; ...
       0      0          0          1];
   
R_y = [cos(pitch)  0   sin(pitch)   0; ...
          0        1       0        0; ...
      -sin(pitch)  0   cos(pitch)   0; ...
          0        0       0        1];
   
R_z = [cos(yaw) -sin(yaw)  0        0; ...
       sin(yaw)  cos(yaw)  0        0; ...
         0           0     1        0; ...
         0           0     0        1];

R = MP_C*R_z*R_y*R_x;

Out = R* ([(L/2);+(W/2);(H/2);1]);
MP_U3_X = Out(1);
MP_U3_Y = Out(2);
MP_U3_Z = Out(3);

== matlab function cable_driven_parallel_robot2022/Target Wrench-Jacobian matrix/Subsystem/Transformer/Transform3 ==
  data: roll input; pitch input; yaw input; MP_X input; MP_Y input; MP_Z input; MP_U4_X output; MP_U4_Y output; MP_U4_Z output; L input; W input; H input
function [MP_U4_X,MP_U4_Y,MP_U4_Z] = fcn(roll,pitch,yaw,MP_X,MP_Y,MP_Z,L,W,H)

MP_C = [1  0  0  MP_X; ... 
        0  1  0  MP_Y; ...
        0  0  1  MP_Z; ...
        0  0  0   1];

R_x = [1      0          0          0; ...
       0  cos(roll) -sin(roll)      0; ...
       0  sin(roll)  cos(roll)      0; ...
       0      0          0          1];
   
R_y = [cos(pitch)  0   sin(pitch)   0; ...
          0        1       0        0; ...
      -sin(pitch)  0   cos(pitch)   0; ...
          0        0       0        1];
   
R_z = [cos(yaw) -sin(yaw)  0        0; ...
       sin(yaw)  cos(yaw)  0        0; ...
         0           0     1        0; ...
         0           0     0        1];

R = MP_C*R_z*R_y*R_x;

Out = R* ([-(L/2);+(W/2);(H/2);1]);
MP_U4_X = Out(1);
MP_U4_Y = Out(2);
MP_U4_Z = Out(3);

== matlab function cable_driven_parallel_robot2022/Target Wrench-Jacobian matrix/Subsystem/Transformer/Transform4 ==
  data: roll input; pitch input; yaw input; MP_X input; MP_Y input; MP_Z input; MP_L1_X output; MP_L1_Y output; MP_L1_Z output; L input; W input; H input
function [MP_L1_X,MP_L1_Y,MP_L1_Z] = fcn(roll, pitch,yaw,MP_X,MP_Y,MP_Z,L,W,H)

MP_C = [1  0  0  MP_X; ... 
        0  1  0  MP_Y; ...
        0  0  1  MP_Z; ...
        0  0  0   1];

R_x = [1      0          0          0; ...
       0  cos(roll) -sin(roll)      0; ...
       0  sin(roll)  cos(roll)      0; ...
       0      0          0          1];
   
R_y = [cos(pitch)  0   sin(pitch)   0; ...
          0        1       0        0; ...
      -sin(pitch)  0   cos(pitch)   0; ...
          0        0       0        1];
   
R_z = [cos(yaw) -sin(yaw)  0        0; ...
       sin(yaw)  cos(yaw)  0        0; ...
         0           0     1        0; ...
         0           0     0        1];

R = MP_C*R_z*R_y*R_x;

Out = R* ([-(L/2);-(W/2) ;-(H/2);1]);
MP_L1_X = Out(1);
MP_L1_Y = Out(2);
MP_L1_Z = Out(3);

== matlab function cable_driven_parallel_robot2022/Target Wrench-Jacobian matrix/Subsystem/Transformer/Transform5 ==
  data: roll input; pitch input; yaw input; MP_X input; MP_Y input; MP_Z input; MP_L2_X output; MP_L2_Y output; MP_L2_Z output; L input; W input; H input
function [MP_L2_X,MP_L2_Y,MP_L2_Z] = fcn(roll,pitch,yaw,MP_X,MP_Y,MP_Z,L,W,H)

MP_C = [1  0  0  MP_X; ... 
        0  1  0  MP_Y; ...
        0  0  1  MP_Z; ...
        0  0  0   1];

R_x = [1      0          0          0; ...
       0  cos(roll) -sin(roll)      0; ...
       0  sin(roll)  cos(roll)      0; ...
       0      0          0          1];
   
R_y = [cos(pitch)  0   sin(pitch)   0; ...
          0        1       0        0; ...
      -sin(pitch)  0   cos(pitch)   0; ...
          0        0       0        1];
   
R_z = [cos(yaw) -sin(yaw)  0        0; ...
       sin(yaw)  cos(yaw)  0        0; ...
         0           0     1        0; ...
         0           0     0        1];

R = MP_C*R_z*R_y*R_x;

Out = R* ([(L/2);-(W/2);-(H/2);1]);
MP_L2_X = Out(1);
MP_L2_Y = Out(2);
MP_L2_Z = Out(3);

== matlab function cable_driven_parallel_robot2022/Target Wrench-Jacobian matrix/Subsystem/Transformer/Transform6 ==
  data: roll input; pitch input; yaw input; MP_X input; MP_Y input; MP_Z input; MP_L3_X output; MP_L3_Y output; MP_L3_Z output; L input; W input; H input
function [MP_L3_X,MP_L3_Y,MP_L3_Z] = fcn(roll,pitch,yaw,MP_X,MP_Y,MP_Z,L,W,H)

MP_C = [1  0  0  MP_X; ... 
        0  1  0  MP_Y; ...
        0  0  1  MP_Z; ...
        0  0  0   1];

R_x = [1      0          0          0; ...
       0  cos(roll) -sin(roll)      0; ...
       0  sin(roll)  cos(roll)      0; ...
       0      0          0          1];
   
R_y = [cos(pitch)  0   sin(pitch)   0; ...
          0        1       0        0; ...
      -sin(pitch)  0   cos(pitch)   0; ...
          0        0       0        1];
   
R_z = [cos(yaw) -sin(yaw)  0        0; ...
       sin(yaw)  cos(yaw)  0        0; ...
         0           0     1        0; ...
         0           0     0        1];

R = MP_C*R_z*R_y*R_x;

Out = R* ([(L/2);+(W/2);-(H/2);1]);
MP_L3_X = Out(1);
MP_L3_Y = Out(2);
MP_L3_Z = Out(3);

== matlab function cable_driven_parallel_robot2022/Target Wrench-Jacobian matrix/Subsystem/Transformer/Transform7 ==
  data: roll input; pitch input; yaw input; MP_X input; MP_Y input; MP_Z input; MP_L4_X output; MP_L4_Y output; MP_L4_Z output; L input; W input; H input
function [MP_L4_X,MP_L4_Y,MP_L4_Z] = fcn(roll,pitch,yaw,MP_X,MP_Y,MP_Z,L,W,H)

MP_C = [1  0  0  MP_X; ... 
        0  1  0  MP_Y; ...
        0  0  1  MP_Z; ...
        0  0  0   1];

R_x = [1      0          0          0; ...
       0  cos(roll) -sin(roll)      0; ...
       0  sin(roll)  cos(roll)      0; ...
       0      0          0          1];
   
R_y = [cos(pitch)  0   sin(pitch)   0; ...
          0        1       0        0; ...
      -sin(pitch)  0   cos(pitch)   0; ...
          0        0       0        1];
   
R_z = [cos(yaw) -sin(yaw)  0        0; ...
       sin(yaw)  cos(yaw)  0        0; ...
         0           0     1        0; ...
         0           0     0        1];

R = MP_C*R_z*R_y*R_x;

Out = R* ([-(L/2);+(W/2);-(H/2);1]);
MP_L4_X = Out(1);
MP_L4_Y = Out(2);
MP_L4_Z = Out(3);

== matlab function cable_driven_parallel_robot2022/Actuators-CableTension-MovingPlatform/Moving Platform/Moving Platform/MATLAB Function ==
  data: u input; y output; rest input
function y = fcn(u,rest)

if rest == 1
    y = 0;
else
    y = u; 
end

== matlab function cable_driven_parallel_robot2022/Actuators-CableTension-MovingPlatform/QuadRotor/Subsystem/Subsystem/MATLAB Function ==
  data: rest0 input; rest output; init0 input; init output
function [rest,init] = fcn(rest0,init0)

if rest0==1
    rest=rest0;
    init=0;
else
  rest = rest0;
  init = init0;

end

== matlab function cable_driven_parallel_robot2022/Actuators-CableTension-MovingPlatform/QuadRotor/Subsystem/Subsystem1/MATLAB Function ==
  data: rest0 input; rest output; init0 input; init output
function [rest,init] = fcn(rest0,init0)

if rest0==1
    rest=rest0;
    init=0;
else
  rest = rest0;
  init = init0;

end

== matlab function cable_driven_parallel_robot2022/Actuators-CableTension-MovingPlatform/Moving Platform/Moving Platform/Subsystem1/MATLAB Function ==
  data: rest0 input; rest output; init0 input; init output
function [rest,init] = fcn(rest0,init0)

if rest0==1
    rest=rest0;
    init=0;
else
  rest = rest0;
  init = init0;

end

== matlab function cable_driven_parallel_robot2022/Target Wrench-Jacobian matrix/Subsystem/MATLAB Function3 ==
  data: T input; T_MP output; MP_Pose input; ME_Pose input; T_ME output
function [T_MP,T_ME] = fcn(T,MP_Pose,ME_Pose)

T_MP = zeros(3,1);

T_MP(1) = ((ME_Pose(1)-MP_Pose(1))/abs(ME_Pose(1)-MP_Pose(1)))*T(1);
T_MP(2) = ((ME_Pose(2)-MP_Pose(2))/abs(ME_Pose(2)-MP_Pose(2)))*T(2);
T_MP(3) = ((ME_Pose(3)-MP_Pose(3))/abs(ME_Pose(3)-MP_Pose(3)))*T(3);

T_ME = zeros(3,1);
T_ME(1) = ((MP_Pose(1)-ME_Pose(1))/abs(MP_Pose(1)-ME_Pose(1)))*T(1);
T_ME(2) = ((MP_Pose(2)-ME_Pose(2))/abs(MP_Pose(2)-ME_Pose(2)))*T(2);
T_ME(3) = ((MP_Pose(3)-ME_Pose(3))/abs(MP_Pose(3)-ME_Pose(3)))*T(3);

if( (ME_Pose(1)-MP_Pose(1)) == 0 )
    T_MP(1)=0;
    T_ME(1)=0;
end

if( (ME_Pose(2)-MP_Pose(2)) == 0 )
    T_MP(2)=0;
    T_ME(2)=0;
end

if( (ME_Pose(3)-MP_Pose(3)) == 0 )
    T_MP(3)=0;
    T_ME(3)=0;
end
